simulink model "HarnessModel_Reducer"  (R2026a)
settings: Solver=daessc  StopTime=100
PreLoadFcn:
  | setupHarness_Reducer
undefined symbols (not defined in the file or in its folder): AxleTorqueInput, MotorTorqueInput
libraries: fl_lib x20, nesl_utility x9
settings Model: Creator=isaacito  LastModifiedBy=isaacito
settings SimscapeCC: SimscapeNominalValues="[{\"value\":\"1\",\"unit\":\"A\"},{\"value\":\"1\",\"unit\":\"bar\"},{\"value\":\"1\",\"unit\":\"cm^2\"},{\"value\":\"1\",\"unit\":\"cm^3/s\"},{\"value\":\"1\",\"unit\":\"kJ/kg\"},{\"value\":\"1\",\"unit\":\"kW\"},{\"value\":\"1\",\"unit\":\"l\"},{\"value\":\"1\",\"unit\":\"N\"},{\"value\":\"1\",\"unit\":\"N*m\"},{\"value\":\"1\",\"unit\":\"V\"}]"  SimscapeLogLimitData=off  SimscapeLogDataHistory=5000.0

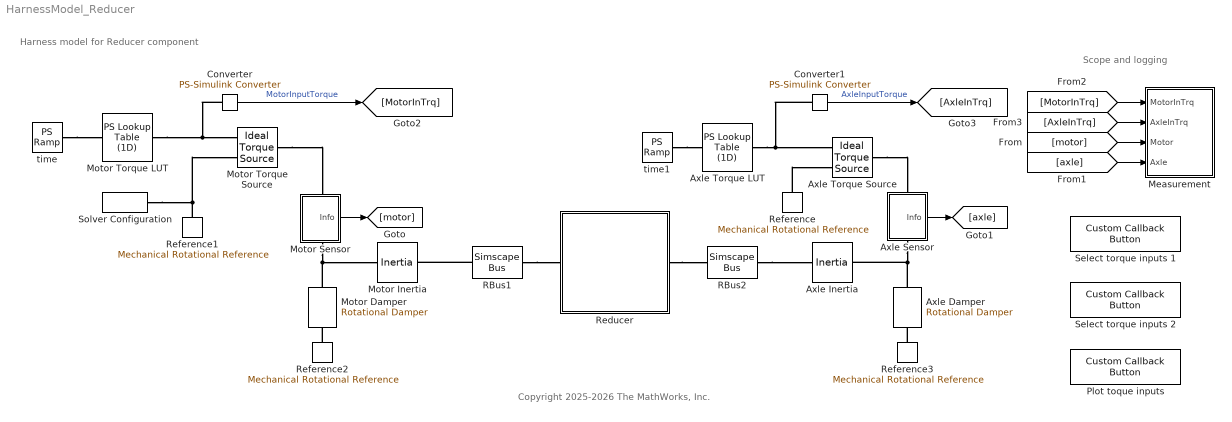
== system HarnessModel_Reducer ==
  note: Scope and logging
  note: Harness model for Reducer component
  note: Copyright 2025-2026 The MathWorks, Inc.
  Axle Damper : fl_lib/Mechanical/Rotational Elements/Rotational Damper  D=0.001 N*m*s/rad  w_specify=off  w_priority=None  w=0 rad/s  w_nominal_specify=off  w_nominal_value=1  w_nominal_unit=rad/s  t_specify=off  t_priority=None  t=0 N*m  t_nominal_specify=off  t_nominal_value=1  t_nominal_unit=N*m
      settings: AttributesFormatString=%<D> %<D_unit>
  Axle Inertia : fl_lib/Mechanical/Rotational Elements/Inertia  inertia=1*0.3^2 kg*m^2  num_ports=foundation.enum.numPorts2.two  w_specify=off  w_priority=High  w=0 rad/s  w_nominal_specify=off  w_nominal_value=1  w_nominal_unit=rad/s  t_specify=off  t_priority=None  t=0 N*m  t_nominal_specify=off  t_nominal_value=1  t_nominal_unit=N*m
      settings: AttributesFormatString=%<inertia> %<inertia_unit>
  Axle Sensor : Subsystem
      settings: PortSchema="{\"entries\":[{\"content\":{\"sides\":[{\"content\":{\"connectorIds\":[\"LConn1\"]},\"type\":\"ConnectorPlacement.EquallySpacedRectSide\",\"uuid\":\"7cb7a15d-af66-48ef-9de9-cdb3b1401e0b\"},{\"content\":{\"connectorIds\":[\"RConn1\"],\"side\":\"RIGHT\"},\"type\":\"ConnectorPlacement.EquallySpacedRectSide\",\"uuid\":\"d5a7816f-d5e7-4c87-ba60-ac5e138dbf88\"},{\"content\":{\"side\":\"TOP\"},\"type\":\"ConnectorPlacement.EquallySpacedRectSide\",\"uuid\":\"e2ba9299-9967-4b5b-86b8-9756387493c3\"},{\"content\":{\"connectorIds\":[\"Out1\"],\"side\":\"BOTTOM\"},\"type\":\"ConnectorPlacement.EquallySpacedRectSide\",\"uuid\":\"625d0ca4-27f8-4dfa-9ab7-6eb306368651\"}]},\"type\":\"ConnectorPlacement.EquallySpacedConnector\",\"uuid\":\"7d3b1d8c-d441-4b58-8085-c9ebd3a2ccac\"}],\"packageUris\":[\"http://schema.mathworks.com/mf0/Connector/R2020b\"],\"version\":\"1.0\"}"
  Axle Torque LUT : fl_lib/Physical Signals/Lookup Tables/PS Lookup Table (1D)  Description=|  x="AxleTorqueInput.Time.value(\"s\") s"  f="AxleTorqueInput.Torque.value(\"N*m\") N*m"  interp_method=simscape.enum.interpolation.smooth  extrap_method=simscape.enum.extrapolation.nearest
      | % This text was automatically added by the Signal Util.
      | % SignalDesignMatrixStart
      | [0, 5, 0; 8, 20, 100; 30, 50, -100; 65, 70, 0]
      | % SignalDesignMatrixEnd
  Axle Torque Source : fl_lib/Mechanical/Mechanical Sources/Ideal Torque Source
  Converter : nesl_utility/PS-Simulink Converter  PhysicalDomain=network_engine_domain  SubClassName=ps_output  LeftPortType=input  RightPortType=output  PseudoPeriodic=off  Frequencies=[]  VectorFormat=inherit  Unit=N*m  AffineConversion=off
  Converter1 : nesl_utility/PS-Simulink Converter  PhysicalDomain=network_engine_domain  SubClassName=ps_output  LeftPortType=input  RightPortType=output  PseudoPeriodic=off  Frequencies=[]  VectorFormat=inherit  Unit=N*m  AffineConversion=off
  Measurement : Subsystem
  Motor Damper : fl_lib/Mechanical/Rotational Elements/Rotational Damper  D=0.01 N*m*s/rad  w_specify=off  w_priority=None  w=0 rad/s  w_nominal_specify=off  w_nominal_value=1  w_nominal_unit=rad/s  t_specify=off  t_priority=None  t=0 N*m  t_nominal_specify=off  t_nominal_value=1  t_nominal_unit=N*m
      settings: AttributesFormatString=%<D> %<D_unit>
  Motor Inertia : fl_lib/Mechanical/Rotational Elements/Inertia  inertia=10*0.3^2 kg*m^2  num_ports=foundation.enum.numPorts2.two  w_specify=off  w_priority=High  w=0 rad/s  w_nominal_specify=off  w_nominal_value=1  w_nominal_unit=rad/s  t_specify=off  t_priority=None  t=0 N*m  t_nominal_specify=off  t_nominal_value=1  t_nominal_unit=N*m
      settings: AttributesFormatString=%<inertia> %<inertia_unit>
  Motor Sensor : Subsystem
      settings: PortSchema="{\"entries\":[{\"content\":{\"sides\":[{\"content\":{\"connectorIds\":[\"LConn1\"]},\"type\":\"ConnectorPlacement.EquallySpacedRectSide\",\"uuid\":\"7cb7a15d-af66-48ef-9de9-cdb3b1401e0b\"},{\"content\":{\"connectorIds\":[\"RConn1\"],\"side\":\"RIGHT\"},\"type\":\"ConnectorPlacement.EquallySpacedRectSide\",\"uuid\":\"d5a7816f-d5e7-4c87-ba60-ac5e138dbf88\"},{\"content\":{\"connectorIds\":[\"Out1\"],\"side\":\"TOP\"},\"type\":\"ConnectorPlacement.EquallySpacedRectSide\",\"uuid\":\"e2ba9299-9967-4b5b-86b8-9756387493c3\"}]},\"type\":\"ConnectorPlacement.EquallySpacedConnector\",\"uuid\":\"7d3b1d8c-d441-4b58-8085-c9ebd3a2ccac\"}],\"packageUris\":[\"http://schema.mathworks.com/mf0/Connector/R2020b\"],\"version\":\"1.0\"}"
  Motor Torque LUT : fl_lib/Physical Signals/Lookup Tables/PS Lookup Table (1D)  Description=|  x="MotorTorqueInput.Time.value(\"s\") s"  f="MotorTorqueInput.Torque.value(\"N*m\") N*m"  interp_method=simscape.enum.interpolation.smooth  extrap_method=simscape.enum.extrapolation.nearest
      | % This text was automatically inserted by Signal Tool.
      | % SignalDesignMatrixStart
      | [0, 3, 0; 4, 5, -50; 6, 10, 50; 12, 13, 0]
      | % SignalDesignMatrixEnd
  Motor Torque Source : fl_lib/Mechanical/Mechanical Sources/Ideal Torque Source
  Plot toque inputs : CustomCallbackButton  Configuration="{\"components\":[{\"name\":\"BackgroundImageComponent\",\"settings\":{\"image\":{\"size\":[0,0],\"src\":\"default\",\"srcOrientation\":\"Right\"},\"position\":[0,0,1,1]}},{\"name\":\"ButtonStateComponent\",\"settings\":{\"buttonType\":\"momentary\",\"clickFcn\":\"bevutil1.SignalUtil.plotLookupTable1DBlocks(gcs, SearchDepth=1)\",\"onValue\":1,\"position\":[0,0,1,1],\"pressDelay\":\"500\",\"pressFcn\":\"\",\"repeatInterval\":\"0\",\"states\":[{\"horizontalAlignment\":\"center\",\"image\":{\"position\":[0,0,1,1],\"size\":[1,1],\"src\":\"default\",\"srcOrientation\":\"Right\"},\"label\":{\"color\":[0.01176470588,0.01176470588,0.01176470588,1],\"icon\":{\"size\":[0,0],\"src\":\"default\",\"srcOrientation\":\"Right\"},\"iconOffset\":0,\"iconPlacement\":\"left\",\"opacity\":1,\"show\":true,\"text\":{\"content\":\"Plot LUTs\",\"font\":\"Helvetica\"}},\"labelOffset\":[0,0],\"verticalAlignment\":\"middle\"},{\"horizontalAlignment\":\"center\",\"image\":{\"position\":[0,0,1,1],\"size\":[1,1],\"src\":\"default\",\"srcOrientation\":\"Right\"},\"label\":{\"color\":[0.01176470588,0.01176470588,0.01176470588,1],\"icon\":{\"size\":[0,0],\"src\":\"default\",\"srcOrientation\":\"Right\"},\"iconOffset\":0,\"iconPlacement\":\"left\",\"opacity\":1,\"show\":true,\"text\":{\"content\":\"Plot LUTs\",\"font\":\"Helvetica\"}},\"labelOffset\":[0,0],\"verticalAlignment\":\"middle\"},{\"horizontalAlignment\":\"center\",\"image\":{\"position\":[0,0,1,1],\"size\":[1,1],\"src\":\"default\",\"srcOrientation\":\"Right\"},\"label\":{\"color\":[0.01176470588,0.01176470588,0.01176470588,1],\"icon\":{\"size\":[0,0],\"src\":\"default\",\"srcOrientation\":\"Right\"},\"iconOffset\":0,\"iconPlacement\":\"left\",\"opacity\":1,\"show\":true,\"text\":{\"content\":\"Plot LUTs\",\"font\":\"Helvetica\"}},\"labelOffset\":[0,0],\"verticalAlignment\":\"middle\"},{\"horizontalAlignment\":\"center\",\"image\":{\"position\":[0,0,1,1],\"size\":[1,1],\"src\":\"default\",\"srcOrientation\":\"Right\"},\"label\":{\"color\":[0.01176470588,0.01176470588,0.01176470588,1],\"icon\":{\"size\":[0,0],\"src\":\"default\",\"srcOrientation\":\"Right\"},\"iconOffset\":0,\"iconPlacement\":\"left\",\"opacity\":1,\"show\":true,\"text\":{\"content\":\"Plot LUTs\",\"font\":\"Helvetica\"}},\"labelOffset\":[0,0],\"verticalAlignment\":\"middle\"}]}},{\"name\":\"ForegroundImageComponent\",\"settings\":{\"image\":{\"size\":[0,0],\"src\":\"default\",\"srcOrientation\":\"Right\"},\"isForeground\":1,\"position\":[0,0,1,1]}}],\"derived\":{\"blockParameters\":{\"AutoActivate\":true,\"ButtonText\":\"Plot LUTs\",\"ButtonType\":\"Momentary\",\"ClickFcn\":\"bevutil1.SignalUtil.plotLookupTable1DBlocks(gcs, SearchDepth=1)\",\"OnValue\":1,\"PressDelay\":\"500\",\"PressFcn\":\"\",\"RepeatInterval\":\"0\",\"fixedAspectRatio\":\"off\"}},\"settings\":{\"BindingType\":\"standalone\",\"autoActivate\":true,\"backgroundColor\":[244,244,244,1],\"backgroundOffset\":0.2,\"backgroundOpacity\":1,\"fixedAspectRatio\":\"off\",\"foregroundColor\":[0.01176470588,0.01176470588,0.01176470588,1],\"migratedFromLegacy\":true,\"useBackgroundColor\":true,\"variant\":\"callback\",\"version\":\"R2025a\"},\"type\":\"Button\"}"  CustomBackgroundColor="{\"color\":[0.9568627451,0.9568627451,0.9568627451],\"show\":true}"
  RBus1 : SimscapeBus  HierarchyStrings=AngSpd  ConnectionType=Bus: Bus_Rotational
      settings: AttributesFormatString=%<ConnectionType>
  RBus2 : SimscapeBus  HierarchyStrings=AngSpd  ConnectionType=Bus: Bus_Rotational
      settings: AttributesFormatString=%<ConnectionType>
  Reducer : Subsystem  ReferencedSubsystem=Reducer_Basic_refsub
      settings: OpenFcn="open_system(gcb, \"force\")"
  Reference{,1..3} (4 alike) : fl_lib/Mechanical/Rotational Elements/Mechanical Rotational Reference
  Select torque inputs 1 : CustomCallbackButton  Configuration="{\"components\":[{\"name\":\"BackgroundImageComponent\",\"settings\":{\"image\":{\"size\":[0,0],\"src\":\"default\",\"srcOrientation\":\"Right\"},\"position\":[0,0,1,1]}},{\"name\":\"ButtonStateComponent\",\"settings\":{\"buttonType\":\"momentary\",\"clickFcn\":\"loadLUTData_Reducer_Motor_Constant\\nloadLUTData_Reducer_Axle_Constant\",\"onValue\":1,\"position\":[0,0,1,1],\"pressDelay\":\"500\",\"pressFcn\":\"\",\"repeatInterval\":\"0\",\"states\":[{\"horizontalAlignment\":\"center\",\"image\":{\"position\":[0,0,1,1],\"size\":[1,1],\"src\":\"default\",\"srcOrientation\":\"Right\"},\"label\":{\"color\":[0.01176470588,0.01176470588,0.01176470588,1],\"icon\":{\"size\":[0,0],\"src\":\"default\",\"srcOrientation\":\"Right\"},\"iconOffset\":0,\"iconPlacement\":\"left\",\"opacity\":1,\"show\":true,\"text\":{\"content\":\"Constant\",\"font\":\"Helvetica\"}},\"labelOffset\":[0,0],\"verticalAlignment\":\"middle\"},{\"horizontalAlignment\":\"center\",\"image\":{\"position\":[0,0,1,1],\"size\":[1,1],\"src\":\"default\",\"srcOrientation\":\"Right\"},\"label\":{\"color\":[0.01176470588,0.01176470588,0.01176470588,1],\"icon\":{\"size\":[0,0],\"src\":\"default\",\"srcOrientation\":\"Right\"},\"iconOffset\":0,\"iconPlacement\":\"left\",\"opacity\":1,\"show\":true,\"text\":{\"content\":\"Constant\",\"font\":\"Helvetica\"}},\"labelOffset\":[0,0],\"verticalAlignment\":\"middle\"},{\"horizontalAlignment\":\"center\",\"image\":{\"position\":[0,0,1,1],\"size\":[1,1],\"src\":\"default\",\"srcOrientation\":\"Right\"},\"label\":{\"color\":[0.01176470588,0.01176470588,0.01176470588,1],\"icon\":{\"size\":[0,0],\"src\":\"default\",\"srcOrientation\":\"Right\"},\"iconOffset\":0,\"iconPlacement\":\"left\",\"opacity\":1,\"show\":true,\"text\":{\"content\":\"Constant\",\"font\":\"Helvetica\"}},\"labelOffset\":[0,0],\"verticalAlignment\":\"middle\"},{\"horizontalAlignment\":\"center\",\"image\":{\"position\":[0,0,1,1],\"size\":[1,1],\"src\":\"default\",\"srcOrientation\":\"Right\"},\"label\":{\"color\":[0.01176470588,0.01176470588,0.01176470588,1],\"icon\":{\"size\":[0,0],\"src\":\"default\",\"srcOrientation\":\"Right\"},\"iconOffset\":0,\"iconPlacement\":\"left\",\"opacity\":1,\"show\":true,\"text\":{\"content\":\"Constant\",\"font\":\"Helvetica\"}},\"labelOffset\":[0,0],\"verticalAlignment\":\"middle\"}]}},{\"name\":\"ForegroundImageComponent\",\"settings\":{\"image\":{\"size\":[0,0],\"src\":\"default\",\"srcOrientation\":\"Right\"},\"isForeground\":1,\"position\":[0,0,1,1]}}],\"derived\":{\"blockParameters\":{\"AutoActivate\":true,\"ButtonText\":\"Constant\",\"ButtonType\":\"Momentary\",\"ClickFcn\":\"loadLUTData_Reducer_Motor_Constant\\nloadLUTData_Reducer_Axle_Constant\",\"OnValue\":1,\"PressDelay\":\"500\",\"PressFcn\":\"\",\"RepeatInterval\":\"0\",\"fixedAspectRatio\":\"off\"}},\"settings\":{\"BindingType\":\"standalone\",\"autoActivate\":true,\"backgroundColor\":[244,244,244,1],\"backgroundOffset\":0.2,\"backgroundOpacity\":1,\"fixedAspectRatio\":\"off\",\"foregroundColor\":[0.01176470588,0.01176470588,0.01176470588,1],\"migratedFromLegacy\":true,\"useBackgroundColor\":true,\"variant\":\"callback\",\"version\":\"R2025a\"},\"type\":\"Button\"}"  CustomBackgroundColor="{\"color\":[0.9568627451,0.9568627451,0.9568627451],\"show\":true}"
  Select torque inputs 2 : CustomCallbackButton  Configuration="{\"components\":[{\"name\":\"BackgroundImageComponent\",\"settings\":{\"image\":{\"size\":[0,0],\"src\":\"default\",\"srcOrientation\":\"Right\"},\"position\":[0,0,1,1]}},{\"name\":\"ButtonStateComponent\",\"settings\":{\"buttonType\":\"momentary\",\"clickFcn\":\"loadLUTData_Reducer_Motor_FlipTorque\\nloadLUTData_Reducer_Axle_FlipTorque\",\"onValue\":1,\"position\":[0,0,1,1],\"pressDelay\":\"500\",\"pressFcn\":\"\",\"repeatInterval\":\"0\",\"states\":[{\"horizontalAlignment\":\"center\",\"image\":{\"position\":[0,0,1,1],\"size\":[1,1],\"src\":\"default\",\"srcOrientation\":\"Right\"},\"label\":{\"color\":[0.01176470588,0.01176470588,0.01176470588,1],\"icon\":{\"size\":[0,0],\"src\":\"default\",\"srcOrientation\":\"Right\"},\"iconOffset\":0,\"iconPlacement\":\"left\",\"opacity\":1,\"show\":true,\"text\":{\"content\":\"Flip\",\"font\":\"Helvetica\"}},\"labelOffset\":[0,0],\"verticalAlignment\":\"middle\"},{\"horizontalAlignment\":\"center\",\"image\":{\"position\":[0,0,1,1],\"size\":[1,1],\"src\":\"default\",\"srcOrientation\":\"Right\"},\"label\":{\"color\":[0.01176470588,0.01176470588,0.01176470588,1],\"icon\":{\"size\":[0,0],\"src\":\"default\",\"srcOrientation\":\"Right\"},\"iconOffset\":0,\"iconPlacement\":\"left\",\"opacity\":1,\"show\":true,\"text\":{\"content\":\"Flip\",\"font\":\"Helvetica\"}},\"labelOffset\":[0,0],\"verticalAlignment\":\"middle\"},{\"horizontalAlignment\":\"center\",\"image\":{\"position\":[0,0,1,1],\"size\":[1,1],\"src\":\"default\",\"srcOrientation\":\"Right\"},\"label\":{\"color\":[0.01176470588,0.01176470588,0.01176470588,1],\"icon\":{\"size\":[0,0],\"src\":\"default\",\"srcOrientation\":\"Right\"},\"iconOffset\":0,\"iconPlacement\":\"left\",\"opacity\":1,\"show\":true,\"text\":{\"content\":\"Flip\",\"font\":\"Helvetica\"}},\"labelOffset\":[0,0],\"verticalAlignment\":\"middle\"},{\"horizontalAlignment\":\"center\",\"image\":{\"position\":[0,0,1,1],\"size\":[1,1],\"src\":\"default\",\"srcOrientation\":\"Right\"},\"label\":{\"color\":[0.01176470588,0.01176470588,0.01176470588,1],\"icon\":{\"size\":[0,0],\"src\":\"default\",\"srcOrientation\":\"Right\"},\"iconOffset\":0,\"iconPlacement\":\"left\",\"opacity\":1,\"show\":true,\"text\":{\"content\":\"Flip\",\"font\":\"Helvetica\"}},\"labelOffset\":[0,0],\"verticalAlignment\":\"middle\"}]}},{\"name\":\"ForegroundImageComponent\",\"settings\":{\"image\":{\"size\":[0,0],\"src\":\"default\",\"srcOrientation\":\"Right\"},\"isForeground\":1,\"position\":[0,0,1,1]}}],\"derived\":{\"blockParameters\":{\"AutoActivate\":true,\"ButtonText\":\"Flip\",\"ButtonType\":\"Momentary\",\"ClickFcn\":\"loadLUTData_Reducer_Motor_FlipTorque\\nloadLUTData_Reducer_Axle_FlipTorque\",\"OnValue\":1,\"PressDelay\":\"500\",\"PressFcn\":\"\",\"RepeatInterval\":\"0\",\"fixedAspectRatio\":\"off\"}},\"settings\":{\"BindingType\":\"standalone\",\"autoActivate\":true,\"backgroundColor\":[244,244,244,1],\"backgroundOffset\":0.2,\"backgroundOpacity\":1,\"fixedAspectRatio\":\"off\",\"foregroundColor\":[0.01176470588,0.01176470588,0.01176470588,1],\"migratedFromLegacy\":true,\"useBackgroundColor\":true,\"variant\":\"callback\",\"version\":\"R2025a\"},\"type\":\"Button\"}"  CustomBackgroundColor="{\"color\":[0.9568627451,0.9568627451,0.9568627451],\"show\":true}"
  Solver Configuration : nesl_utility/Solver Configuration  PhysicalDomain=network_engine_domain  SubClassName=solver  LeftPortType=input  RightPortType=generic  Tones=[]  Harmonics=[]  SimulateNoise=off  Profile=off  UseLocalSampling=off  EnableSwitchedLinearOptims=on  FrequencyDomain=off  UseCCode=off  RelTol=0.001  AbsTol=0.001  MinStep=1e-09  ToWorkspace=off  RevertToSquareIcSolve=off  NumHomotopyIterations=100  PhasorMode=off  PhasorModeNumHarmonics=1  ConsistencySolver=NEWTON_XTOL_AFTER_FTOL  CanonicalOrdering=UNORDERED  OptimizeIntermediates=UNOPTIMIZED  IndexReductionMethod=DerivativeReplacement  DoDC=off  ResidualTolerance=1e-09  ConsistencyTolSource=GLOBAL  ConsistencyAbsTol=0.001  ConsistencyRelTol=0.001  ConsistencyTolFactor=0.001  UseLocalSolver=off  LocalSolverChoice=NE_BACKWARD_EULER_ADVANCER  ResolveIndetEquations=on  FunctionEvalNumThread=1  LocalSolverSampleTime=0.001  DoFixedCost=off  MaxNonlinIter=3  MaxModeIter=2  ComputeImpulses=off  ImpulseIterations=2  LinearAlgebra=auto  LinearAlgebraNumThread=0  EquationFormulation=NE_TIME_EF  DelaysMemoryBudget=1024  AutomaticFiltering=on  FilteringTimeConstant=0.001  PartitionStorageMethod=AS_NEEDED  PartitionMemoryBudget=1024  PartitionMethod=ROBUST  MultibodyUseLocalSolver=off  MultibodyLocalSolverChoice=ODE1  MultibodyLocalSolverSampleTime=0.001
      settings: AttributesFormatString=Local solver: %<UseLocalSolver>
  time : fl_lib/Physical Signals/Sources/PS Ramp  slope=1  start_time=0 s  initial_output=0 s  ZeroCross=true
  time1 : fl_lib/Physical Signals/Sources/PS Ramp  slope=1  start_time=0 s  initial_output=0 s  ZeroCross=true
  wires:
  [motor] -> Measurement/3(Motor)
  [axle] -> Measurement/4(Axle)
  [MotorInTrq] -> Measurement/1(MotorInTrq)
  [AxleInTrq] -> Measurement/2(AxleInTrq)
  Converter/1 -> [MotorInTrq]  "MotorInputTorque"
  Motor Sensor/1(Info) -> [motor]
  Converter1/1 -> [AxleInTrq]  "AxleInputTorque"
  Axle Sensor/1(Info) -> [axle]
  connections:
  Converter/LConn1 -- Motor Torque Source/RConn1 -- Motor Torque LUT/RConn1
  time/RConn1 -- Motor Torque LUT/LConn1
  Reference1/LConn1 -- Solver Configuration/RConn1 -- Motor Torque Source/RConn2
  Motor Torque Source/LConn1 -- Motor Sensor/LConn1
  RBus1/LConn1 -- Motor Inertia/LConn1
  Motor Sensor/RConn1 -- Motor Inertia/RConn1 -- Motor Damper/LConn1
  Reference2/LConn1 -- Motor Damper/RConn1
  RBus1/RConn1 -- Reducer/LConn1
  Converter1/LConn1 -- Axle Torque Source/RConn1 -- Axle Torque LUT/RConn1
  time1/RConn1 -- Axle Torque LUT/LConn1
  Reference/LConn1 -- Axle Torque Source/RConn2
  Axle Sensor/LConn1 -- Axle Inertia/RConn1 -- Axle Damper/LConn1
  RBus2/LConn1 -- Axle Inertia/LConn1
  Reference3/LConn1 -- Axle Damper/RConn1
  Reducer/RConn1 -- RBus2/RConn1
  Axle Torque Source/LConn1 -- Axle Sensor/RConn1

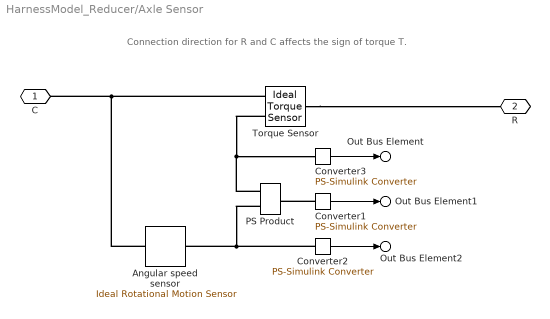
== system HarnessModel_Reducer/Axle Sensor ==
  note: Connection direction for R and C affects the sign of torque T.
  Angular speed sensor : fl_lib/Mechanical/Mechanical Sensors/Ideal Rotational Motion Sensor  reference=foundation.enum.MeasurementReference.absolute  acceleration_port=false  velocity_port=true  position_port=false  wrap_angle=false  offset=0 rad
  Converter1 : nesl_utility/PS-Simulink Converter  PhysicalDomain=network_engine_domain  SubClassName=ps_output  LeftPortType=input  RightPortType=output  PseudoPeriodic=off  Frequencies=[]  VectorFormat=inherit  Unit=W  AffineConversion=off
  Converter2 : nesl_utility/PS-Simulink Converter  PhysicalDomain=network_engine_domain  SubClassName=ps_output  LeftPortType=input  RightPortType=output  PseudoPeriodic=off  Frequencies=[]  VectorFormat=inherit  Unit=rpm  AffineConversion=off
  Converter3 : nesl_utility/PS-Simulink Converter  PhysicalDomain=network_engine_domain  SubClassName=ps_output  LeftPortType=input  RightPortType=output  PseudoPeriodic=off  Frequencies=[]  VectorFormat=inherit  Unit=N*m  AffineConversion=off
  PS Product : fl_lib/Physical Signals/Functions/PS Product
  Torque Sensor : fl_lib/Mechanical/Mechanical Sensors/Ideal Torque Sensor
  C : PMIOPort  Side=Left  ConnectionType=Connection: foundation.mechanical.rotational.rotational
  R : PMIOPort  Port=2  Side=Right  ConnectionType=Connection: foundation.mechanical.rotational.rotational
  Out Bus Element : Outport  PortName=Info  Element=Torque
  Out Bus Element1 : Outport  PortName=Info  Element=Power
  Out Bus Element2 : Outport  PortName=Info  Element=AngularSpeed
  wires:
  Converter1/1 -> Out Bus Element1/1
  Converter3/1 -> Out Bus Element/1
  Converter2/1 -> Out Bus Element2/1
  connections:
  Converter2/LConn1 -- PS Product/LConn2 -- Angular speed sensor/RConn1
  Torque Sensor/RConn2 -- PS Product/LConn1 -- Converter3/LConn1
  Torque Sensor/RConn1 -- C/RConn1 -- Angular speed sensor/LConn1
  Torque Sensor/LConn1 -- R/RConn1
  Converter1/LConn1 -- PS Product/RConn1

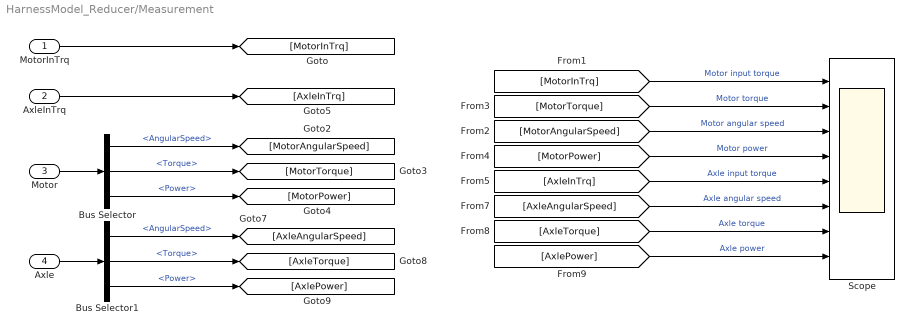
== system HarnessModel_Reducer/Measurement ==
  MotorInTrq : Inport
  AxleInTrq : Inport  Port=2
  Motor : Inport  Port=3
  Axle : Inport  Port=4
  Bus Selector : BusSelector  OutputSignals=AngularSpeed,Torque,Power
  Bus Selector1 : BusSelector  OutputSignals=AngularSpeed,Torque,Power
  Scope : Scope  NumInputPorts=8
      settings: ActiveDisplayString=6  ActiveDisplayYMinimum=-162.26108623058525  ActiveDisplayYMaximum=420.3303836183369
  wires:
  Motor/1 -> Bus Selector/1
  Axle/1 -> Bus Selector1/1
  MotorInTrq/1 -> [MotorInTrq]
  Bus Selector/1 -> [MotorAngularSpeed]  "<AngularSpeed>"
  Bus Selector/2 -> [MotorTorque]  "<Torque>"
  Bus Selector/3 -> [MotorPower]  "<Power>"
  Bus Selector1/1 -> [AxleAngularSpeed]  "<AngularSpeed>"
  Bus Selector1/2 -> [AxleTorque]  "<Torque>"
  Bus Selector1/3 -> [AxlePower]  "<Power>"
  AxleInTrq/1 -> [AxleInTrq]
  [AxlePower] -> Scope/8  "Axle power"
  [AxleTorque] -> Scope/7  "Axle torque"
  [MotorInTrq] -> Scope/1  "Motor input torque"
  [MotorTorque] -> Scope/2  "Motor torque"
  [MotorAngularSpeed] -> Scope/3  "Motor angular speed"
  [MotorPower] -> Scope/4  "Motor power"
  [AxleInTrq] -> Scope/5  "Axle input torque"
  [AxleAngularSpeed] -> Scope/6  "Axle angular speed"

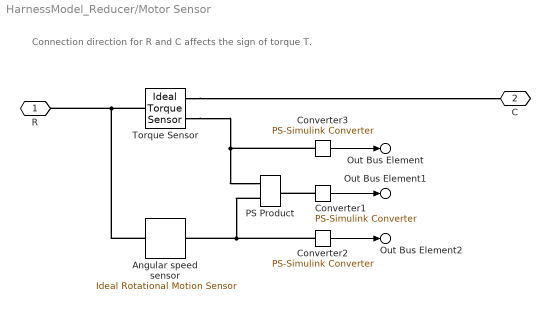
== system HarnessModel_Reducer/Motor Sensor ==
  note: Connection direction for R and C affects the sign of torque T.
  Angular speed sensor : fl_lib/Mechanical/Mechanical Sensors/Ideal Rotational Motion Sensor  reference=foundation.enum.MeasurementReference.absolute  acceleration_port=false  velocity_port=true  position_port=false  wrap_angle=false  offset=0 rad
  Converter1 : nesl_utility/PS-Simulink Converter  PhysicalDomain=network_engine_domain  SubClassName=ps_output  LeftPortType=input  RightPortType=output  PseudoPeriodic=off  Frequencies=[]  VectorFormat=inherit  Unit=W  AffineConversion=off
  Converter2 : nesl_utility/PS-Simulink Converter  PhysicalDomain=network_engine_domain  SubClassName=ps_output  LeftPortType=input  RightPortType=output  PseudoPeriodic=off  Frequencies=[]  VectorFormat=inherit  Unit=rpm  AffineConversion=off
  Converter3 : nesl_utility/PS-Simulink Converter  PhysicalDomain=network_engine_domain  SubClassName=ps_output  LeftPortType=input  RightPortType=output  PseudoPeriodic=off  Frequencies=[]  VectorFormat=inherit  Unit=N*m  AffineConversion=off
  PS Product : fl_lib/Physical Signals/Functions/PS Product
  Torque Sensor : fl_lib/Mechanical/Mechanical Sensors/Ideal Torque Sensor
  R : PMIOPort  Side=Left  ConnectionType=Connection: foundation.mechanical.rotational.rotational
  C : PMIOPort  Port=2  Side=Right  ConnectionType=Connection: foundation.mechanical.rotational.rotational
  Out Bus Element : Outport  PortName=Info  Element=Torque
  Out Bus Element1 : Outport  PortName=Info  Element=Power
  Out Bus Element2 : Outport  PortName=Info  Element=AngularSpeed
  wires:
  Converter1/1 -> Out Bus Element1/1
  Converter3/1 -> Out Bus Element/1
  Converter2/1 -> Out Bus Element2/1
  connections:
  Converter2/LConn1 -- PS Product/LConn2 -- Angular speed sensor/RConn1
  Angular speed sensor/LConn1 -- Torque Sensor/LConn1 -- R/RConn1
  Converter1/LConn1 -- PS Product/RConn1
  Torque Sensor/RConn2 -- Converter3/LConn1 -- PS Product/LConn1
  Torque Sensor/RConn1 -- C/RConn1
